simulink model "FlyingFluxFOC"  (R2026b)
settings: Solver=FixedStepDiscrete  StopTime=experimentCfg.Duration  FixedStep=bridgeCfg.Ts
PostLoadFcn:
  | addpath(fullfile(fileparts(get_param(bdroot,'FileName')),'..','build_process'));initialize_flying_foc(bdroot);
model workspace (MAT data in the model file):
  bridgeCfg.Rs = 0.5
  bridgeCfg.Ld = 0.001
  bridgeCfg.Lq = 0.001
  bridgeCfg.Flux = 0.035
  bridgeCfg.PolePairs = 4
  bridgeCfg.J = 0.0005
  bridgeCfg.B = 0.0001
  bridgeCfg.Id0 = 0
  bridgeCfg.Iq0 = 0
  bridgeCfg.Speed0 = 80
  bridgeCfg.Position0 = 0.1
  bridgeCfg.Ts = 5e-06
  bridgeCfg.Vdc = 48
  bridgeCfg.DiodeVf = 0.7
  bridgeCfg.DiodeRon = 0.01
  bridgeCfg.MechanicalEnabled = 1
  bridgeCfg.CurrentTolerance = 1e-09
  bridgeCfg.VoltageTolerance = 1e-08
  bridgeCfg.MaxCurrent = 200
  bridgeCfg.MaxSpeed = 1000
  bridgeCfg.MaxAngleStep = 0.1
  bridgeCfg.State0 = [0; 0; 80; 0.1]
  bridgeCfg.Vector = [5e-06; 0.5; 0.001; 0.001; 0.035; 4; 0.0005; 0.0001; 48; 0.7; 0.01; 1; 1e-09; 1e-08; 200; 1000; 0.1]
  currentCfg.Ts = 5e-05
  currentCfg.BandwidthHz = 500
  currentCfg.Kpd = 3.14159265359
  currentCfg.Kpq = 3.14159265359
  currentCfg.Kid = 1570.79632679
  currentCfg.Kiq = 1570.79632679
  currentCfg.Kaw = 20000
  experimentCfg.Duration = 1
  experimentCfg.SpeedReference = 100
  experimentCfg.LoadTorque = 0
  experimentCfg.LoadTime = 0.5
  experimentCfg.Enable = 1
  experimentCfg.ResetTime = Inf
  experimentCfg.ResetDuration = 0.005
  experimentCfg.DisableTime = Inf
  experimentCfg.ReenableTime = Inf
  experimentCfg.ObserverOffTime = Inf
  experimentCfg.ObserverOnTime = Inf
  fluxCfg.Ts = 5e-05
  fluxCfg.Rs = 0.5
  fluxCfg.L = 0.001
  fluxCfg.Flux = 0.035
  fluxCfg.PolePairs = 4
  fluxCfg.LeakEnable = 1
  fluxCfg.LeakHz = 10
  fluxCfg.DcEnable = 1
  fluxCfg.DcHz = 3
  fluxCfg.FrequencyHz = 5
  fluxCfg.MinCompOmega = 20
  fluxCfg.FullCompOmega = 100
  fluxCfg.MaxCompGain = 4
  fluxCfg.MinFlux = 0.015
  fluxCfg.MaxFlux = 0.0525
  fluxCfg.MinOmega = 120
  fluxCfg.MaxResidual = 5
  fluxCfg.LeakA = 0.996863336985
  fluxCfg.LeakB = 4.99215423658e-05
  fluxCfg.DcA = 0.999057966197
  fluxCfg.FrequencyA = 0.998430436728
  flyingCfg.Ts = 5e-05
  flyingCfg.PolePairs = 4
  flyingCfg.MinOmega = 140
  flyingCfg.MaxResidual = 5
  flyingCfg.CaptureTime = 0.025
  flyingCfg.PrechargeTime = 0.01
  flyingCfg.LossTime = 0.001
  flyingCfg.Timeout = 0.6
  flyingCfg.CaptureCurrentMax = 0.5
  flyingCfg.CaptureVoltageMax = 23.9438703638
  flyingCfg.CurrentTrip = 12
  flyingCfg.SpeedKp = 0.08
  flyingCfg.SpeedKi = 0.8
  flyingCfg.SpeedKaw = 20
  flyingCfg.CurrentMax = 8
  flyingCfg.CurrentReferenceSlew = 100
  flyingCfg.Vector = [5e-05; 4; 140; 5; 500; 200; 20; 12000; 0.5; 23.9438703638; 12; 0.08; 0.8; 20; 8; 100]
  flyingStim.time = [0 5e-05 0.0001 0.00015 0.0002 0.00025 0.0003 0.00035 0.0004 0.00045 0.0005 0.00055 ... (20001 elements, 20001x1)]
  flyingStim.signals.values = [100 100 100 100 100 100 100 100 100 100 100 100 ... (100005 elements, 20001x5)]
  flyingStim.signals.dimensions = 5
  inverterCfg.Vdc = 48
  inverterCfg.MinDuty = 0.02
  inverterCfg.PwmTs = 5e-05
  inverterCfg.LinearLimit = 26.6043004043
  pllCfg.Ts = 5e-05
  pllCfg.NaturalFrequency = 40
  pllCfg.Damping = 0.707
  pllCfg.Kp = 355.376960974
  pllCfg.Ki = 63165.468167
  pllCfg.Kaw = 502.654824574
  pllCfg.OmegaMax = 1500
  pllCfg.MinMagnitude = 0.015
  pllCfg.LockError = 0.12
  pllCfg.LockSamples = 100
  pllCfg.Theta0 = 0
  pllCfg.Omega0 = 0
libraries: ClarkePark x3, CurrentControl x2, Inverter x1, FluxObserver x1, PMSMBridgePlant x1
settings Model: Creator=24322  LastModifiedBy=24322

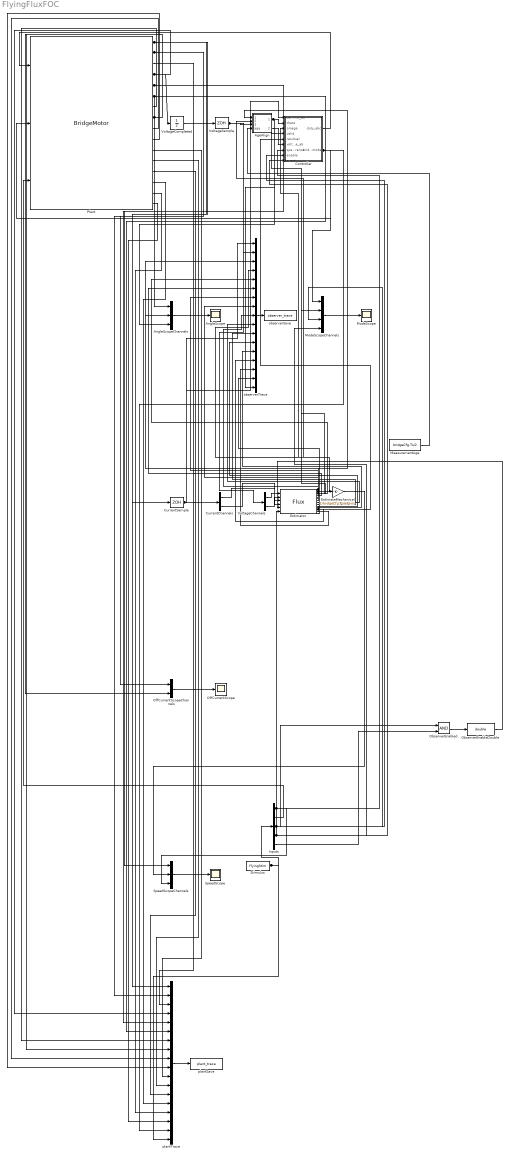
== system FlyingFluxFOC ==
  AgeAlign : MATLAB Function  TreatAsAtomicUnit=on
  AngleScope : Scope
  AngleScopeChannels : Mux  Inputs=3
  Controller : Subsystem
  CurrentChannels : Demux  Outputs=2
  CurrentSample : ZeroOrderHold  SampleTime=currentCfg.Ts
  EstimateMechanical : Gain  Gain=1/bridgeCfg.PolePairs
  Estimator : FluxObserver/Flux  cfg=fluxCfg  trackerCfg=pllCfg
  Inputs : Demux  Outputs=5
  MeasurementAge : Constant  Value=bridgeCfg.Ts/2
  ModeScope : Scope
  ModeScopeChannels : Mux
  ObserverEnableDouble : DataTypeConversion  OutDataTypeStr=double  SaturateOnIntegerOverflow=off  RndMeth=Floor
  ObserverEnabled : Logic  IconShape=distinctive  AllPortsSameDT=off  OutDataTypeStr=boolean
  OffCurrentScope : Scope
  OffCurrentScopeChannels : Mux  Inputs=2
  Plant : PMSMBridgePlant/BridgeMotor  cfg=bridgeCfg
  SpeedScope : Scope
  SpeedScopeChannels : Mux  Inputs=3
  Stimulus : FromWorkspace  VariableName=flyingStim  SampleTime=currentCfg.Ts  Interpolate=off  OutputAfterFinalValue=Holding final value
  VoltageChannels : Demux  Outputs=2
  VoltageCompleted : UnitDelay  InitialCondition=zeros(2,1)  SampleTime=bridgeCfg.Ts
  VoltageSample : ZeroOrderHold  SampleTime=currentCfg.Ts
  observerSave : ToWorkspace  VariableName=observer_trace  SaveFormat=Structure With Time  SampleTime=currentCfg.Ts
  observerTrace : Mux  Inputs=17
  plantSave : ToWorkspace  VariableName=plant_trace  SaveFormat=Structure With Time  SampleTime=currentCfg.Ts
  plantTrace : Mux  Inputs=18
  wires:
  ModeScopeChannels/1 -> ModeScope/1
  OffCurrentScopeChannels/1 -> OffCurrentScope/1
  EstimateMechanical/1 -> SpeedScopeChannels/2
  SpeedScopeChannels/1 -> SpeedScope/1
  AngleScopeChannels/1 -> AngleScope/1
  Estimator/14 -> observerTrace/16
  Estimator/13 -> observerTrace/15
  Estimator/11 -> observerTrace/13
  Estimator/10 -> observerTrace/12
  Estimator/9 -> observerTrace/11
  Estimator/8 -> observerTrace/10
  Estimator/7 -> observerTrace/9
  Estimator/6 -> observerTrace/8
  Estimator/5 -> observerTrace/7
  Estimator/4 -> observerTrace/6
  observerTrace/1 -> observerSave/1
  Plant/16 -> plantTrace/16
  Plant/15 -> plantTrace/15
  Plant/14 -> plantTrace/14
  Plant/13 -> plantTrace/13
  Plant/12 -> plantTrace/12
  Plant/11 -> plantTrace/11
  Plant/10 -> plantTrace/10
  Plant/9 -> plantTrace/9
  Plant/8 -> OffCurrentScopeChannels/2, plantTrace/8
  Plant/7 -> plantTrace/7
  Plant/6 -> AngleScopeChannels/1, plantTrace/6
  Plant/5 -> SpeedScopeChannels/1, plantTrace/5
  Plant/3 -> plantTrace/3
  Plant/2 -> OffCurrentScopeChannels/1, plantTrace/2
  plantTrace/1 -> plantSave/1
  Inputs/1 -> SpeedScopeChannels/3, Controller/7(speed_reference)
  AgeAlign/2(voltage) -> Controller/6(voltage_ab)
  Estimator/12 -> observerTrace/14, Controller/5(residual)
  Estimator/3 -> ModeScopeChannels/2, observerTrace/5, Controller/4(valid)
  AgeAlign/1(theta) -> AngleScopeChannels/3, observerTrace/17, Controller/2(theta)
  MeasurementAge/1 -> AgeAlign/4(age)
  Estimator/2 -> observerTrace/4, EstimateMechanical/1, Controller/3(omega), AgeAlign/2(omega)
  Estimator/1 -> AngleScopeChannels/2, observerTrace/3, AgeAlign/1(rawTheta)
  Inputs/4 -> ModeScopeChannels/4, Controller/9(reset), Estimator/6
  ObserverEnableDouble/1 -> Estimator/5
  ObserverEnabled/1 -> ObserverEnableDouble/1
  Inputs/5 -> ObserverEnabled/2
  Inputs/3 -> ModeScopeChannels/3, Controller/8(enable), ObserverEnabled/1
  CurrentChannels/2 -> Estimator/4
  CurrentChannels/1 -> Estimator/3
  VoltageChannels/2 -> Estimator/2
  VoltageChannels/1 -> Estimator/1
  VoltageSample/1 -> observerTrace/2, AgeAlign/3(measuredVoltage), VoltageChannels/1
  CurrentSample/1 -> observerTrace/1, Controller/1(current_ab), CurrentChannels/1
  VoltageCompleted/1 -> VoltageSample/1
  Plant/4 -> plantTrace/4, VoltageCompleted/1
  Plant/1 -> plantTrace/1, CurrentSample/1
  Inputs/2 -> Plant/3
  Controller/2(bridge_mode) -> ModeScopeChannels/1, Plant/2, plantTrace/17
  Controller/1(duty_abc) -> Plant/1
  Stimulus/1 -> plantTrace/18, Inputs/1

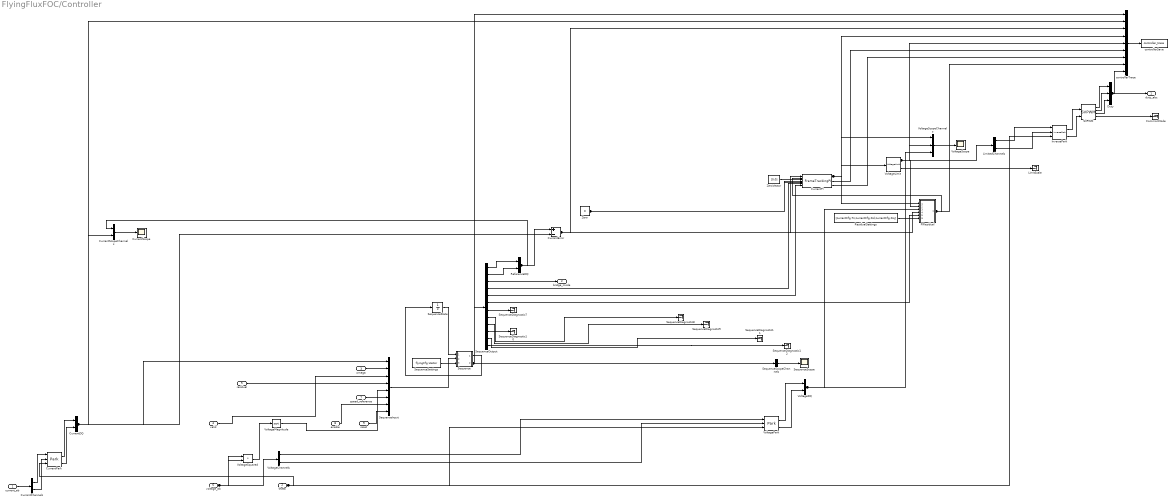
== system FlyingFluxFOC/Controller ==
  current_ab : Inport  OutDataTypeStr=double  PortDimensions=2  SampleTime=currentCfg.Ts
  theta : Inport  Port=2  OutDataTypeStr=double  PortDimensions=1  SampleTime=currentCfg.Ts
  omega : Inport  Port=3  OutDataTypeStr=double  PortDimensions=1  SampleTime=currentCfg.Ts
  valid : Inport  Port=4  OutDataTypeStr=double  PortDimensions=1  SampleTime=currentCfg.Ts
  residual : Inport  Port=5  OutDataTypeStr=double  PortDimensions=1  SampleTime=currentCfg.Ts
  voltage_ab : Inport  Port=6  OutDataTypeStr=double  PortDimensions=2  SampleTime=currentCfg.Ts
  speed_reference : Inport  Port=7  OutDataTypeStr=double  PortDimensions=1  SampleTime=currentCfg.Ts
  enable : Inport  Port=8  OutDataTypeStr=double  PortDimensions=1  SampleTime=currentCfg.Ts
  reset : Inport  Port=9  OutDataTypeStr=double  PortDimensions=1  SampleTime=currentCfg.Ts
  CommonMode : Terminator
  CurrentChannels : Demux  Outputs=2
  CurrentDQ : Mux  Inputs=2
  CurrentError : Sum  Inputs=+-
  CurrentPI : CurrentControl/FrameTrackingPI  currentCfg=currentCfg
  CurrentPark : ClarkePark/Park  SystemSampleTime=-1  VariantActivationTime=update diagram  EmptyChoice=off  PassThrough=off  PassThroughVariantControl=(default)  EmptyChoiceVariantControl=(default)  AllowFlexibleInterface=on  Latency=0  AutoFrameSizeCalculation=off
  CurrentScope : Scope
  CurrentScopeChannels : Mux  Inputs=2
  Duty : Mux  Inputs=3
  InversePark : ClarkePark/InversePark  SystemSampleTime=-1  VariantActivationTime=update diagram  EmptyChoice=off  PassThrough=off  PassThroughVariantControl=(default)  EmptyChoiceVariantControl=(default)  AllowFlexibleInterface=on  Latency=0  AutoFrameSizeCalculation=off
  LimitScale : Terminator
  LimitedChannels : Demux  Outputs=2
  PIResidual : MATLAB Function  TreatAsAtomicUnit=on
  ReferenceDQ : Mux  Inputs=2
  ResidualSettings : Constant  Value=[currentCfg.Ts;currentCfg.Kid;currentCfg.Kiq]
  SVPWM : Inverter/SVPWM  SystemSampleTime=-1  VariantActivationTime=update diagram  EmptyChoice=off  PassThrough=off  PassThroughVariantControl=(default)  EmptyChoiceVariantControl=(default)  AllowFlexibleInterface=on  Latency=0  AutoFrameSizeCalculation=off
  Sequence : MATLAB Function  TreatAsAtomicUnit=on
  SequenceDiagnostic{7..12} (6 alike) : Terminator
  SequenceInput : Mux  Inputs=8
  SequenceOutput : Demux  Outputs=12
  SequenceScope : Scope
  SequenceScopeChannels : Mux  Inputs=1
  SequenceSettings : Constant  Value=flyingCfg.Vector
  SequenceState : UnitDelay  InitialCondition=zeros(8,1)  SampleTime=currentCfg.Ts
  VoltageChannels : Demux  Outputs=2
  VoltageDQ : Mux  Inputs=2
  VoltageLimit : CurrentControl/VoltageLimit  SystemSampleTime=-1  VariantActivationTime=update diagram  EmptyChoice=off  PassThrough=off  PassThroughVariantControl=(default)  EmptyChoiceVariantControl=(default)  AllowFlexibleInterface=on  Latency=0  AutoFrameSizeCalculation=off
  VoltageMagnitude : Sqrt
  VoltagePark : ClarkePark/Park  SystemSampleTime=-1  VariantActivationTime=update diagram  EmptyChoice=off  PassThrough=off  PassThroughVariantControl=(default)  EmptyChoiceVariantControl=(default)  AllowFlexibleInterface=on  Latency=0  AutoFrameSizeCalculation=off
  VoltageScope : Scope
  VoltageScopeChannels : Mux  Inputs=3
  VoltageSquared : DotProduct  OutDataTypeStr=Inherit: Inherit via internal rule
  Zero : Constant  Value=0
  ZeroVector : Constant  Value=[0;0]
  controllerSave : ToWorkspace  VariableName=controller_trace  SaveFormat=Structure With Time  SampleTime=currentCfg.Ts
  controllerTrace : Mux  Inputs=9
  duty_abc : Outport  PortDimensions=3
  bridge_mode : Outport  Port=2  PortDimensions=1
  wires:
  SequenceScopeChannels/1 -> SequenceScope/1
  VoltageScopeChannels/1 -> VoltageScope/1
  CurrentScopeChannels/1 -> CurrentScope/1
  CurrentPI/3 -> controllerTrace/7
  CurrentPI/2 -> controllerTrace/6
  controllerTrace/1 -> controllerSave/1
  SequenceOutput/12 -> SequenceDiagnostic12/1
  SequenceOutput/11 -> SequenceDiagnostic11/1
  SequenceOutput/10 -> SequenceDiagnostic10/1
  SequenceOutput/9 -> SequenceDiagnostic9/1
  SequenceOutput/8 -> SequenceDiagnostic8/1
  SequenceOutput/7 -> SequenceDiagnostic7/1
  Duty/1 -> duty_abc/1, controllerTrace/9
  VoltageLimit/2 -> LimitScale/1
  SVPWM/4 -> CommonMode/1
  SVPWM/3 -> Duty/3
  SVPWM/2 -> Duty/2
  SVPWM/1 -> Duty/1
  InversePark/2 -> SVPWM/2
  InversePark/1 -> SVPWM/1
  LimitedChannels/2 -> InversePark/2
  LimitedChannels/1 -> InversePark/1
  ResidualSettings/1 -> PIResidual/6(settings)
  SequenceOutput/6 -> PIResidual/5(precharge)
  VoltageDQ/1 -> VoltageScopeChannels/3, PIResidual/3(passiveVoltage)
  VoltageLimit/1 -> VoltageScopeChannels/2, controllerTrace/5, LimitedChannels/1, PIResidual/2(limited)
  CurrentPI/1 -> VoltageScopeChannels/1, controllerTrace/4, VoltageLimit/1, PIResidual/1(request)
  SequenceOutput/5 -> CurrentPI/7
  SequenceOutput/4 -> CurrentPI/6
  Zero/1 -> CurrentPI/5, CurrentPI/4
  ZeroVector/1 -> CurrentPI/3
  PIResidual/1(residual) -> controllerTrace/8, CurrentPI/2
  CurrentError/1 -> controllerTrace/3, PIResidual/4(error), CurrentPI/1
  ReferenceDQ/1 -> CurrentScopeChannels/1, CurrentError/1
  SequenceOutput/3 -> bridge_mode/1
  SequenceOutput/2 -> ReferenceDQ/2
  SequenceOutput/1 -> ReferenceDQ/1
  Sequence/2(output) -> SequenceScopeChannels/1, SequenceOutput/1, controllerTrace/1
  Sequence/1(next) -> SequenceState/1
  SequenceSettings/1 -> Sequence/3(parameter)
  SequenceInput/1 -> Sequence/2(input)
  SequenceState/1 -> Sequence/1(state)
  reset/1 -> SequenceInput/8
  enable/1 -> SequenceInput/7
  speed_reference/1 -> SequenceInput/6
  VoltageMagnitude/1 -> SequenceInput/5
  residual/1 -> SequenceInput/4
  valid/1 -> SequenceInput/3
  omega/1 -> SequenceInput/2
  CurrentDQ/1 -> CurrentScopeChannels/2, controllerTrace/2, SequenceInput/1, CurrentError/2
  VoltageSquared/1 -> VoltageMagnitude/1
  VoltagePark/2 -> VoltageDQ/2
  VoltagePark/1 -> VoltageDQ/1
  CurrentPark/2 -> CurrentDQ/2
  CurrentPark/1 -> CurrentDQ/1
  VoltageChannels/2 -> VoltagePark/2
  VoltageChannels/1 -> VoltagePark/1
  theta/1 -> InversePark/3, VoltagePark/3, CurrentPark/3
  CurrentChannels/2 -> CurrentPark/2
  CurrentChannels/1 -> CurrentPark/1
  voltage_ab/1 -> VoltageSquared/2, VoltageSquared/1, VoltageChannels/1
  current_ab/1 -> CurrentChannels/1

== matlab function FlyingFluxFOC/Controller/PIResidual ==
  data: request input; residual output; limited input; passiveVoltage input; error input; precharge input; settings input
function residual=flying_pi_residual(request,limited,passiveVoltage,error,precharge,settings)
%FLYING_PI_RESIDUAL Prepare PI while off, or use actuator feasibility while on.
%#codegen
residual=limited-request;
if precharge>0.5
    % With Kaw=1/Ts this makes I[k+1]=passiveVoltage-P[k].
    residual=passiveVoltage-request-settings(1)*settings(2:3).*error;
end
end

== matlab function FlyingFluxFOC/Controller/Sequence ==
  data: state input; next output; input input; parameter input; output output
function [next,output]=flying_capture_step(state,input,parameter)
%FLYING_CAPTURE_STEP App sequence, using measured dq currents and estimates.
%#codegen
% state=[mode;qualificationN;stageN;lossN;fault;speedI;referenceD;referenceQ].
% input=[id;iq;omegaE;valid;fluxResidual;voltageMagnitude;speedRefM;enable;reset].
% output=[idRef;iqRef;bridgeMode;piEnable;piReset;precharge;mode;fault;
%         qualificationN;lossN;speedI;iqTarget]. No plant truth is an input.
p=cast(parameter,'like',state);u=cast(input,'like',state);
next=state;output=zeros(12,1,'like',state);mode=state(1);
if u(8)<0.5 || u(9)>0.5
    next(:)=0;output(5)=1;return
end
if ~all(isfinite(u))
    next(:)=0;next(1)=5;next(5)=7;output(5)=1;output(7)=5;output(8)=7;return
end
output(7:11)=[mode;state(5);state(2);state(4);state(6)];
if mode==5,output(5)=1;return,end
if mode==0,next(1)=1;output(5)=1;return,end
current=hypot(u(1),u(2));speedError=u(7)-u(3)/p(2);
healthy=u(4)>0.5 && abs(u(3))>=p(3) && u(5)>=0 && u(5)<=p(4);
output(4)=1;
if mode==1 || mode==2
    % PWM remains off while PI total voltage follows passive terminal voltage.
    output(1:2)=u(1:2);output(6)=1;
    next(6)=-p(12)*speedError;next(7:8)=u(1:2);
    if mode==1
        next(3)=state(3)+1;
        if healthy,next(2)=min(state(2)+1,p(5));else,next(2)=0;end
        if next(2)>=p(5)
            if u(7)*u(3)<=0,next(1)=5;next(5)=2;
            elseif u(6)>p(10),next(1)=5;next(5)=3;
            elseif current>p(9),next(1)=5;next(5)=4;
            else,next(1)=2;next(3)=0;next(4)=0;end
        elseif next(3)>=p(8),next(1)=5;next(5)=1;
        end
    else
        if healthy,next(4)=0;next(3)=state(3)+1;
        else,next(4)=state(4)+1;next(3)=0;end
        if healthy && u(7)*u(3)<=0,next(1)=5;next(5)=2;
        elseif u(6)>p(10),next(1)=5;next(5)=3;
        elseif current>p(9),next(1)=5;next(5)=4;
        elseif next(4)>=p(7),next(1)=5;next(5)=5;
        elseif next(3)>=p(6),next(1)=3;end
    end
elseif mode==3
    output(1:2)=state(7:8);output(3)=1;
    iqRaw=p(12)*speedError+state(6);
    iqTarget=min(max(iqRaw,-p(15)),p(15));output(12)=iqTarget;
    step=p(1)*p(16);
    next(7)=state(7)+min(max(-state(7),-step),step);
    next(8)=state(8)+min(max(iqTarget-state(8),-step),step);
    next(6)=state(6)+p(1)*(p(13)*speedError+p(14)*(state(8)-iqRaw));
    if healthy,next(4)=0;else,next(4)=state(4)+1;end
    if healthy && u(7)*u(3)<=0,next(1)=5;next(5)=2;
    elseif next(4)>=p(7),next(1)=5;next(5)=5;end
else
    next(1)=5;next(5)=7;
end
if current>p(11),next(1)=5;next(5)=6;end
end

== matlab function FlyingFluxFOC/AgeAlign ==
  data: rawTheta input; theta output; omega input; measuredVoltage input; age input; voltage output
function [theta,voltage]=flying_angle_align(rawTheta,omega,measuredVoltage,age)
%FLYING_ANGLE_ALIGN First-order age compensation of completed-interval sample.
%#codegen
advance=omega*age;theta=atan2(sin(rawTheta+advance),cos(rawTheta+advance));
c=cos(advance);s=sin(advance);
voltage=[c*measuredVoltage(1)-s*measuredVoltage(2); ...
    s*measuredVoltage(1)+c*measuredVoltage(2)];
end
